simulink model "furuta_block_model_pi"  (R2026b)
settings: Solver=ode14x  StopTime=5  FixedStep=driveElectrical.sampleTime
model workspace (MAT data in the model file):
  controlPeriod = 0.01
  driveElectrical.R = 0.41
  driveElectrical.L = 0.00051
  driveElectrical.Ke = 1.73002596752
  driveElectrical.sampleTime = 0.0001
  driveElectrical.Kp = 0.480663675999
  driveElectrical.Ki = 386.415896392
  furutaPPOAgent : rl.agent.rlPPOAgent (value not decoded)
  furutaSACAgent : rl.agent.rlSACAgent (value not decoded)
  furutaToolboxMpc = mpc
  furutaToolboxMpc.Ts = 0.01
  furutaToolboxMpc.PredictionHorizon = 20
  furutaToolboxMpc.ControlHorizon = 20
  furutaToolboxMpc.Model.Plant = ss
  furutaToolboxMpc.Model.Plant.InputName_ = "MV1"
  furutaToolboxMpc.Model.Plant.InputGroup_.Manipulated = 1
  furutaToolboxMpc.Model.Plant.OutputName_ = ["MO1"; "MO2"; "MO3"; "MO4"; "MO5"; "MO6"; "MO7"; "MO8"]
  furutaToolboxMpc.Model.Plant.OutputGroup_.Measured = [1 2 3 4 5 6 7 8]
  furutaToolboxMpc.Model.Plant.IOSize_ = [8 1]
  furutaToolboxMpc.Model.Plant.Data_ = ltipack.ssdata
  furutaToolboxMpc.Model.Plant.Data_.a = [1  -0.00902674267589  0.00993774320897  -2.4767657698e-05; 0  1.0129802947  5.33054368483e-05  0.0100355972733; 0  -1.80504476453  0.987560350231  -0.00796081332398; 0  2.59780112786  0.0106592935191  1.01144622057]
  furutaToolboxMpc.Model.Plant.Data_.c = [1  0  0  0; 0  1  0  0; 0  0  1  0; 0  0  0  1; 23.187012799  50.483540443  3.96076595787  4.74600329341; 0  69.1342012244  4.52520194197  5.64653884547; 0  0  1.92549619263  1.610475723; 0  0  0  1.43133536407]
  furutaToolboxMpc.Model.Plant.Data_.dx0 = [0; 0; 0; 0]
  furutaToolboxMpc.Model.Plant.Data_.x0 = [0; 0; 0; 0]
  furutaToolboxMpc.Model.Plant.Data_.b = [0.0186770373086; -0.0159916310545; 3.73189493068; -3.19778805573]
  furutaToolboxMpc.Model.Plant.Data_.d = [0; 0; 0; 0; 0; 0; 0; 0]
  furutaToolboxMpc.Model.Plant.Data_.u0 = 0
  furutaToolboxMpc.Model.Plant.Data_.y0 = [0; 0; 0; 0; 0; 0; 0; 0]
  furutaToolboxMpc.Model.Plant.Data_.Delay.Input = 0
  furutaToolboxMpc.Model.Plant.Data_.Delay.Output = [0; 0; 0; 0; 0; 0; 0; 0]
  furutaToolboxMpc.Model.Plant.Data_.Delay.Internal = []
  furutaToolboxMpc.Model.Plant.Data_.Ts = 0.01
  furutaToolboxMpc.Model.Disturbance = []
  furutaToolboxMpc.Model.Noise = []
  furutaToolboxMpc.Model.Nominal.X = [0; 0; 0; 0]
  furutaToolboxMpc.Model.Nominal.DX = [0; 0; 0; 0]
  furutaToolboxMpc.Model.Nominal.U = 0
  furutaToolboxMpc.Model.Nominal.Y = [0; 0; 0; 0; 0; 0; 0; 0]
  furutaToolboxMpc.ManipulatedVariables.Min = [-1; -1; -1; -1; -1; -1; -1; -1; -1; -1; -1; -1; -1; -1; -1; -1; -1; -1; -1; -1]
  furutaToolboxMpc.ManipulatedVariables.Max = [1; 1; 1; 1; 1; 1; 1; 1; 1; 1; 1; 1; 1; 1; 1; 1; 1; 1; 1; 1]
  furutaToolboxMpc.ManipulatedVariables.MinECR = [0; 0; 0; 0; 0; 0; 0; 0; 0; 0; 0; 0; 0; 0; 0; 0; 0; 0; 0; 0]
  furutaToolboxMpc.ManipulatedVariables.MaxECR = [0; 0; 0; 0; 0; 0; 0; 0; 0; 0; 0; 0; 0; 0; 0; 0; 0; 0; 0; 0]
  furutaToolboxMpc.ManipulatedVariables.RateMin = -Inf
  furutaToolboxMpc.ManipulatedVariables.RateMax = Inf
  furutaToolboxMpc.ManipulatedVariables.RateMinECR = 0
  furutaToolboxMpc.ManipulatedVariables.RateMaxECR = 0
  furutaToolboxMpc.ManipulatedVariables.Target = 'nominal'
  furutaToolboxMpc.ManipulatedVariables.Name = 'MV1'
  furutaToolboxMpc.ManipulatedVariables.Units = ''
  furutaToolboxMpc.ManipulatedVariables.ScaleFactor = 1
  furutaToolboxMpc.ManipulatedVariables.Type = 'continuous'
  furutaToolboxMpc.OutputVariables(1).Min = [-Inf; -Inf; -Inf; -Inf; -Inf; -Inf; -Inf; -Inf; -Inf; -Inf; -Inf; -Inf; -Inf; -Inf; -Inf; -Inf; -Inf; -Inf; -Inf; -Inf]
  furutaToolboxMpc.OutputVariables(1).Max = [Inf; Inf; Inf; Inf; Inf; Inf; Inf; Inf; Inf; Inf; Inf; Inf; Inf; Inf; Inf; Inf; Inf; Inf; Inf; Inf]
  furutaToolboxMpc.OutputVariables(1).MinECR = [2; 2; 2; 2; 2; 2; 2; 2; 2; 2; 2; 2; 2; 2; 2; 2; 2; 2; 2; 2]
  furutaToolboxMpc.OutputVariables(1).MaxECR = [2; 2; 2; 2; 2; 2; 2; 2; 2; 2; 2; 2; 2; 2; 2; 2; 2; 2; 2; 2]
  furutaToolboxMpc.OutputVariables(1).Name = 'MO1'
  furutaToolboxMpc.OutputVariables(1).Units = ''
  furutaToolboxMpc.OutputVariables(1).ScaleFactor = 1
  furutaToolboxMpc.OutputVariables(2).Min = [-Inf; -Inf; -Inf; -Inf; -Inf; -Inf; -Inf; -Inf; -Inf; -Inf; -Inf; -Inf; -Inf; -Inf; -Inf; -Inf; -Inf; -Inf; -Inf; -Inf]
  furutaToolboxMpc.OutputVariables(2).Max = [Inf; Inf; Inf; Inf; Inf; Inf; Inf; Inf; Inf; Inf; Inf; Inf; Inf; Inf; Inf; Inf; Inf; Inf; Inf; Inf]
  furutaToolboxMpc.OutputVariables(2).MinECR = [2; 2; 2; 2; 2; 2; 2; 2; 2; 2; 2; 2; 2; 2; 2; 2; 2; 2; 2; 2]
  furutaToolboxMpc.OutputVariables(2).MaxECR = [2; 2; 2; 2; 2; 2; 2; 2; 2; 2; 2; 2; 2; 2; 2; 2; 2; 2; 2; 2]
  furutaToolboxMpc.OutputVariables(2).Name = 'MO2'
  furutaToolboxMpc.OutputVariables(2).Units = ''
  furutaToolboxMpc.OutputVariables(2).ScaleFactor = 1
  furutaToolboxMpc.OutputVariables(3).Min = [-Inf; -Inf; -Inf; -Inf; -Inf; -Inf; -Inf; -Inf; -Inf; -Inf; -Inf; -Inf; -Inf; -Inf; -Inf; -Inf; -Inf; -Inf; -Inf; -Inf]
  furutaToolboxMpc.OutputVariables(3).Max = [Inf; Inf; Inf; Inf; Inf; Inf; Inf; Inf; Inf; Inf; Inf; Inf; Inf; Inf; Inf; Inf; Inf; Inf; Inf; Inf]
  furutaToolboxMpc.OutputVariables(3).MinECR = [2; 2; 2; 2; 2; 2; 2; 2; 2; 2; 2; 2; 2; 2; 2; 2; 2; 2; 2; 2]
  furutaToolboxMpc.OutputVariables(3).MaxECR = [2; 2; 2; 2; 2; 2; 2; 2; 2; 2; 2; 2; 2; 2; 2; 2; 2; 2; 2; 2]
  furutaToolboxMpc.OutputVariables(3).Name = 'MO3'
  furutaToolboxMpc.OutputVariables(3).Units = ''
  furutaToolboxMpc.OutputVariables(3).ScaleFactor = 1
  furutaToolboxMpc.OutputVariables(4).Min = [-Inf; -Inf; -Inf; -Inf; -Inf; -Inf; -Inf; -Inf; -Inf; -Inf; -Inf; -Inf; -Inf; -Inf; -Inf; -Inf; -Inf; -Inf; -Inf; -Inf]
  furutaToolboxMpc.OutputVariables(4).Max = [Inf; Inf; Inf; Inf; Inf; Inf; Inf; Inf; Inf; Inf; Inf; Inf; Inf; Inf; Inf; Inf; Inf; Inf; Inf; Inf]
  furutaToolboxMpc.OutputVariables(4).MinECR = [2; 2; 2; 2; 2; 2; 2; 2; 2; 2; 2; 2; 2; 2; 2; 2; 2; 2; 2; 2]
  furutaToolboxMpc.OutputVariables(4).MaxECR = [2; 2; 2; 2; 2; 2; 2; 2; 2; 2; 2; 2; 2; 2; 2; 2; 2; 2; 2; 2]
  furutaToolboxMpc.OutputVariables(4).Name = 'MO4'
  furutaToolboxMpc.OutputVariables(4).Units = ''
  furutaToolboxMpc.OutputVariables(4).ScaleFactor = 1
  furutaToolboxMpc.OutputVariables(5).Min = [-Inf; -Inf; -Inf; -Inf; -Inf; -Inf; -Inf; -Inf; -Inf; -Inf; -Inf; -Inf; -Inf; -Inf; -Inf; -Inf; -Inf; -Inf; -Inf; -Inf]
  furutaToolboxMpc.OutputVariables(5).Max = [Inf; Inf; Inf; Inf; Inf; Inf; Inf; Inf; Inf; Inf; Inf; Inf; Inf; Inf; Inf; Inf; Inf; Inf; Inf; Inf]
  furutaToolboxMpc.OutputVariables(5).MinECR = [2; 2; 2; 2; 2; 2; 2; 2; 2; 2; 2; 2; 2; 2; 2; 2; 2; 2; 2; 2]
  furutaToolboxMpc.OutputVariables(5).MaxECR = [2; 2; 2; 2; 2; 2; 2; 2; 2; 2; 2; 2; 2; 2; 2; 2; 2; 2; 2; 2]
  furutaToolboxMpc.OutputVariables(5).Name = 'MO5'
  furutaToolboxMpc.OutputVariables(5).Units = ''
  furutaToolboxMpc.OutputVariables(5).ScaleFactor = 1
  furutaToolboxMpc.OutputVariables(6).Min = [-Inf; -Inf; -Inf; -Inf; -Inf; -Inf; -Inf; -Inf; -Inf; -Inf; -Inf; -Inf; -Inf; -Inf; -Inf; -Inf; -Inf; -Inf; -Inf; -Inf]
  furutaToolboxMpc.OutputVariables(6).Max = [Inf; Inf; Inf; Inf; Inf; Inf; Inf; Inf; Inf; Inf; Inf; Inf; Inf; Inf; Inf; Inf; Inf; Inf; Inf; Inf]
  furutaToolboxMpc.OutputVariables(6).MinECR = [2; 2; 2; 2; 2; 2; 2; 2; 2; 2; 2; 2; 2; 2; 2; 2; 2; 2; 2; 2]
  furutaToolboxMpc.OutputVariables(6).MaxECR = [2; 2; 2; 2; 2; 2; 2; 2; 2; 2; 2; 2; 2; 2; 2; 2; 2; 2; 2; 2]
  furutaToolboxMpc.OutputVariables(6).Name = 'MO6'
  furutaToolboxMpc.OutputVariables(6).Units = ''
  furutaToolboxMpc.OutputVariables(6).ScaleFactor = 1
  furutaToolboxMpc.OutputVariables(7).Min = [-Inf; -Inf; -Inf; -Inf; -Inf; -Inf; -Inf; -Inf; -Inf; -Inf; -Inf; -Inf; -Inf; -Inf; -Inf; -Inf; -Inf; -Inf; -Inf; -Inf]
  furutaToolboxMpc.OutputVariables(7).Max = [Inf; Inf; Inf; Inf; Inf; Inf; Inf; Inf; Inf; Inf; Inf; Inf; Inf; Inf; Inf; Inf; Inf; Inf; Inf; Inf]
  furutaToolboxMpc.OutputVariables(7).MinECR = [2; 2; 2; 2; 2; 2; 2; 2; 2; 2; 2; 2; 2; 2; 2; 2; 2; 2; 2; 2]
  furutaToolboxMpc.OutputVariables(7).MaxECR = [2; 2; 2; 2; 2; 2; 2; 2; 2; 2; 2; 2; 2; 2; 2; 2; 2; 2; 2; 2]
  furutaToolboxMpc.OutputVariables(7).Name = 'MO7'
  furutaToolboxMpc.OutputVariables(7).Units = ''
  furutaToolboxMpc.OutputVariables(7).ScaleFactor = 1
  furutaToolboxMpc.OutputVariables(8).Min = [-Inf; -Inf; -Inf; -Inf; -Inf; -Inf; -Inf; -Inf; -Inf; -Inf; -Inf; -Inf; -Inf; -Inf; -Inf; -Inf; -Inf; -Inf; -Inf; -Inf]
  furutaToolboxMpc.OutputVariables(8).Max = [Inf; Inf; Inf; Inf; Inf; Inf; Inf; Inf; Inf; Inf; Inf; Inf; Inf; Inf; Inf; Inf; Inf; Inf; Inf; Inf]
  furutaToolboxMpc.OutputVariables(8).MinECR = [2; 2; 2; 2; 2; 2; 2; 2; 2; 2; 2; 2; 2; 2; 2; 2; 2; 2; 2; 2]
  furutaToolboxMpc.OutputVariables(8).MaxECR = [2; 2; 2; 2; 2; 2; 2; 2; 2; 2; 2; 2; 2; 2; 2; 2; 2; 2; 2; 2]
  furutaToolboxMpc.OutputVariables(8).Name = 'MO8'
  furutaToolboxMpc.OutputVariables(8).Units = ''
  furutaToolboxMpc.OutputVariables(8).ScaleFactor = 1
  furutaToolboxMpc.Weights.ManipulatedVariables = [1; 1; 1; 1; 1; 1; 1; 1; 1; 1; 1; 1; 1; 1; 1; 1; 1; 1; 1; 1]
  furutaToolboxMpc.Weights.ManipulatedVariablesRate = 1e-05
  furutaToolboxMpc.Weights.OutputVariables = [3.16227766017  3.16227766017  1  1  0  0  0  0; 3.16227766017  3.16227766017  1  1  0  0  0  0; 3.16227766017  3.16227766017  1  1  0  0  0  0; 3.16227766017  3.16227766017  1  1  0  0  0  0; 3.16227766017  3.16227766017  1  1  0  0  0  0; 3.16227766017  3.16227766017  1  1  0  0  0  0; 3.16227766017  3.16227766017  1  1  0  0  0  0; 3.16227766017  3.16227766017  1  1  0  0  0  0; 3.16227766017  3.16227766017  1  1  0  0  0  0; 3.16227766017  3.16227766017  1  1  0  0  0  0; 3.16227766017  3.16227766017  1  1  0  0  0  0; 3.16227766017  3.16227766017  1  1  0  0  0  0; 3.16227766017  3.16227766017  1  1  0  0  0  0; 3.16227766017  3.16227766017  1  1  0  0  0  0; 3.16227766017  3.16227766017  1  1  0  0  0  0; 3.16227766017  3.16227766017  1  1  0  0  0  0; 3.16227766017  3.16227766017  1  1  0  0  0  0; 3.16227766017  3.16227766017  1  1  0  0  0  0; 3.16227766017  3.16227766017  1  1  0  0  0  0; 0  0  0  0  1  1  1  1]
  furutaToolboxMpc.Weights.ECR = 100000
  furutaToolboxMpc.Optimizer.OptimizationType = 'QP'
  furutaToolboxMpc.Optimizer.Solver = 'active-set'
  furutaToolboxMpc.Optimizer.SolverOptions = mpc.solver.options.qp.ActiveSet
  furutaToolboxMpc.Optimizer.SolverOptions.SolverName = 'ActiveSet'
  furutaToolboxMpc.Optimizer.MinOutputECR = 0
  furutaToolboxMpc.Optimizer.UseSuboptimalSolution = 0
  furutaToolboxMpc.Optimizer.CustomSolver = 0
  furutaToolboxMpc.Optimizer.CustomSolverCodeGen = 0
  furutaToolboxMpc.History = [2026 11 18 15 19 42.726]
  furutaToolboxMpc.MPCData = mpcdata
  furutaToolboxMpc.MPCData.IsDirty = 1
  furutaToolboxMpc.MPCData.Ts = 0.01
  furutaToolboxMpc.MPCData.p = 20
  furutaToolboxMpc.MPCData.m = 20
  furutaToolboxMpc.MPCData.UseActiveSetSolver = 1
  furutaToolboxMpc.MPCData.UseSuboptimalSolution = 0
  furutaToolboxMpc.MPCData.CustomSolver = 0
  furutaToolboxMpc.MPCData.CustomSolverCodeGen = 0
  furutaToolboxMpc.MPCData.IsCustomEstimation = 1
  furutaToolboxMpc.MPCData.Uscale = 1
  furutaToolboxMpc.MPCData.Yscale = [1; 1; 1; 1; 1; 1; 1; 1]
  furutaToolboxMpc.MPCData.mvindex = 1
  furutaToolboxMpc.MPCData.myindex = [1; 2; 3; 4; 5; 6; 7; 8]
  furutaToolboxMpc.MPCData.ASOptions.MaxIterations = 120
  furutaToolboxMpc.MPCData.ASOptions.MaxTime = Inf
  furutaToolboxMpc.MPCData.ASOptions.ConstraintTolerance = 1e-06
  furutaToolboxMpc.MPCData.ASOptions.UseWarmStart = 1
  furutaToolboxMpc.MPCData.IPOptions.MaxIterations = 50
  furutaToolboxMpc.MPCData.IPOptions.MaxTime = Inf
  furutaToolboxMpc.MPCData.IPOptions.ConstraintTolerance = 1e-06
  furutaToolboxMpc.MPCData.IPOptions.OptimalityTolerance = 1e-06
  furutaToolboxMpc.MPCData.IPOptions.ComplementarityTolerance = 1e-08
  furutaToolboxMpc.MPCData.IPOptions.StepTolerance = 1e-08
  furutaToolboxMpc.MPCData.ADOptions.AbsoluteTolerance = 0.001
  furutaToolboxMpc.MPCData.ADOptions.RelativeTolerance = 0.001
  furutaToolboxMpc.MPCData.ADOptions.MaxIterations = 1000
  furutaToolboxMpc.MPCData.ADOptions.MaxTime = Inf
  furutaToolboxMpc.MPCData.ADOptions.RelaxationParameter = 1.6
  furutaToolboxMpc.MPCData.ADOptions.PenaltyParameter = 0.1
  furutaToolboxMpc.MPCData.ADOptions.StepSize = 1e-06
  furutaToolboxMpc.MPCData.ADOptions.PrimalInfeasibilityTolerance = 0.0001
  furutaToolboxMpc.MPCData.ADOptions.DualInfeasibilityTolerance = 0.0001
  furutaToolboxMpc.MPCData.ADOptions.EnablePolish = 0
  furutaToolboxMpc.MPCData.ADOptions.PolishRegularization = 1e-06
  furutaToolboxMpc.MPCData.ADOptions.PolishTolerance = 1e-08
  furutaToolboxMpc.MPCData.ADOptions.PolishMaxIterations = 3
  furutaToolboxMpc.MPCData.MIQPOptions.MaxIterations = 1000
  furutaToolboxMpc.MPCData.MIQPOptions.MaxTime = Inf
  furutaToolboxMpc.MPCData.MIQPOptions.ConstraintTolerance = 1e-06
  furutaToolboxMpc.MPCData.MIQPOptions.UseWarmStart = 0
  furutaToolboxMpc.MPCData.MIQPOptions.DiscreteConstraintTolerance = 1e-06
  furutaToolboxMpc.MPCData.MIQPOptions.RoundingAtRootNode = 1
  furutaToolboxMpc.MPCData.MIQPOptions.MaxPendingNodes = 1000
  furutaToolboxMpc.IsEmpty = 0
  furutaToolboxMpc.OldOVIntegrator = {[]; []; []; []; []; []; []; []}
  furutaToolboxMpc.EstGain = 'custom'
  furutaToolboxMpc.OutDistModel = ss
  furutaToolboxMpc.OutDistModel.IOSize_ = [8 1]
  furutaToolboxMpc.OutDistModel.Data_ = ltipack.ssdata
  furutaToolboxMpc.OutDistModel.Data_.d = [0; 0; 0; 0; 0; 0; 0; 0]
  furutaToolboxMpc.OutDistModel.Data_.u0 = 0
  furutaToolboxMpc.OutDistModel.Data_.y0 = [0; 0; 0; 0; 0; 0; 0; 0]
  furutaToolboxMpc.OutDistModel.Data_.Delay.Input = 0
  furutaToolboxMpc.OutDistModel.Data_.Delay.Output = [0; 0; 0; 0; 0; 0; 0; 0]
  furutaToolboxMpc.OutDistModel.Data_.Delay.Internal = []
  furutaToolboxMpc.OutDistModel.Data_.Ts = 0
  furutaToolboxMpc.Version = '26.2'
  initialState = [0; 0.174532925199; 0; 0]
  integrationStep = 0.002
  lqrGain = [-0.560244322113 -7.30813603654 -0.304541725168 -0.68699829167]
  maxTorque = 0.03
  piReplayEnabled = 0
  piReplayState = [0  0  0  0  0; 5  0  0  0  0]
  pidGains = [7.30813603654 0.68699829167 0.560244322113 0.304541725168 0.01]
  plantCoefficients = [0.00019818 0.00016078 0.00016134 0.00013805 0.016934 0.0001 1e-05 0]
  rlRewardLevel = 2
  rmd.model = 'RMD-X6-P20-60-E'
  rmd.voltage = 48
  rmd.gearRatio = 19.612
  rmd.ratedTorque = 20
  rmd.ratedCurrent = 9.5
  rmd.ratedSpeedRPM = 153
  rmd.noLoadSpeedRPM = 176
  rmd.Kt = 2.1
  rmd.currentLSB = 0.01
  rmdCommandDelaySamples = 0
  scenarioStimulus = [0 0.0075 0.0175 0.0275 0.0375 0.0475 0.0575 0.0675 0.0775 0.0875 0.0975 0.1075 ... (2004 elements, 501x4)]
  usePolicyCallback = 0
  useRmd = 1
values from neighbouring files (symbols this model uses):
  C = [B A*B A^2*B A^3*B]    [build_furuta_rmd.m]
  N = 20    [build_furuta_rl.m]    (also in design_classical.m)
  s = load(matFile,'ds')    [analyze_pi_current_run.m]    (also in analyze_pi_speed_run.m; build_furuta_rl.m = sin(x(2));"; build_furuta_simulink.m = s(1); design_classical.m = furuta_scenarios)
  source = [step '/1']    [add_furuta_plant_blocks.m]    (also in build_furuta_pi.m = get_param(line,'SrcPortHandle'); build_furuta_pi_hardware.m = 'Drive interlocks/3'; compare_furuta_actuators.m = get_param([harness '/Requested torque'],'PortHandles'))
  Z = expm([A B; zeros(1,5)]*p.Ts)    [furuta_linearize.m]
undefined symbols (not defined in the file or in its folder): lmpcF, lmpcH, poleGain, sgn, X, Y
libraries: sm_lib x36, nesl_utility x8, fl_lib x7, rllib x2, mpclib x1, slpidlib x1, ee_lib x1
(part 1 of 4)
settings Model: Creator=Lsh  LastModifiedBy=Lsh
settings SimscapeCC: SimscapeLogType=all  SimscapeNominalValues="[{\"value\":\"1\",\"unit\":\"A\"},{\"value\":\"1\",\"unit\":\"bar\"},{\"value\":\"1\",\"unit\":\"cm^2\"},{\"value\":\"1\",\"unit\":\"cm^3/s\"},{\"value\":\"1\",\"unit\":\"kJ/kg\"},{\"value\":\"1\",\"unit\":\"kW\"},{\"value\":\"1\",\"unit\":\"l\"},{\"value\":\"1\",\"unit\":\"N\"},{\"value\":\"1\",\"unit\":\"N*m\"},{\"value\":\"1\",\"unit\":\"V\"},{\"value\":\"0.001\",\"unit\":\"Wb\"}]"  SimscapeUseEnergyAccounting=off

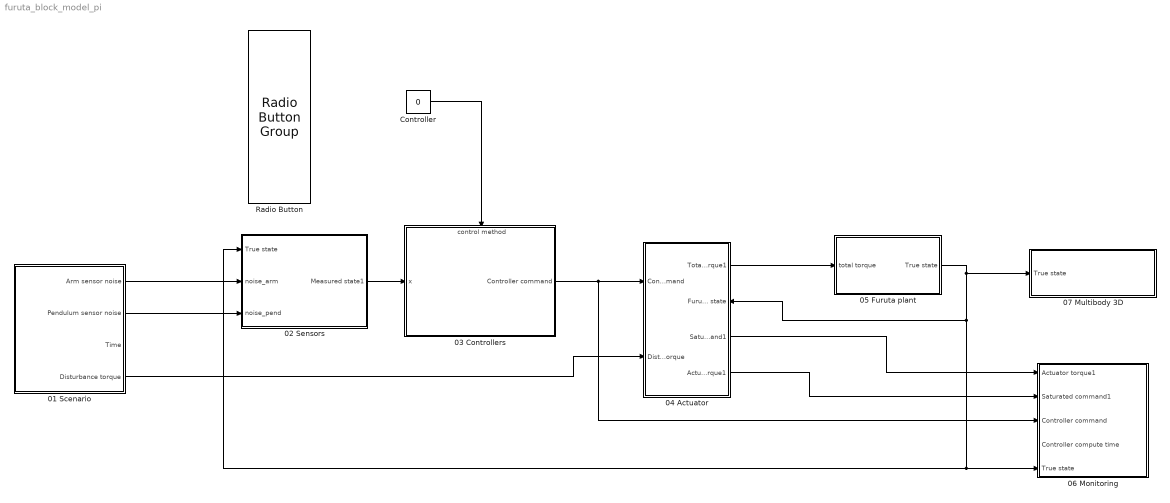
== system furuta_block_model_pi ==
  01 Scenario : Subsystem
  02 Sensors : Subsystem
  03 Controllers : Subsystem
      settings: PortSchema="{\"entries\":[{\"content\":{\"sides\":[{\"content\":{\"connectorIds\":[\"In1\"]},\"type\":\"ConnectorPlacement.EquallySpacedRectSide\",\"uuid\":\"e4b36115-6a1d-4962-9ef8-ed5f31cfcc6a\"},{\"content\":{\"connectorIds\":[\"Out1\"],\"side\":\"RIGHT\"},\"type\":\"ConnectorPlacement.EquallySpacedRectSide\",\"uuid\":\"30852384-c2a0-433b-a443-149c1bfb4c73\"},{\"content\":{\"connectorIds\":[\"In2\"],\"side\":\"TOP\"},\"type\":\"ConnectorPlacement.EquallySpacedRectSide\",\"uuid\":\"d3eba7d3-47d6-4151-b089-0f7eaff5c42c\"},{\"content\":{\"side\":\"BOTTOM\"},\"type\":\"ConnectorPlacement.EquallySpacedRectSide\",\"uuid\":\"8130c781-304c-497e-8c63-b3eca62ccf99\"}]},\"type\":\"ConnectorPlacement.EquallySpacedConnector\",\"uuid\":\"c7c0857b-c1c9-4543-82a8-21998e0f16d7\"}],\"packageUris\":[\"http://schema.mathworks.com/mf0/Connector/R2020b\"],\"version\":\"1.0\"}"
  04 Actuator : Subsystem
      settings: PortSchema="{\"entries\":[{\"content\":{\"sides\":[{\"content\":{\"connectorIds\":[\"In1\",\"In2\"]},\"type\":\"ConnectorPlacement.EquallySpacedRectSide\",\"uuid\":\"dd482a63-174b-40e1-9b64-24dbfdc3f8fa\"},{\"content\":{\"connectorIds\":[\"Out1\",\"In3\",\"Out2\",\"Out3\"],\"side\":\"RIGHT\"},\"type\":\"ConnectorPlacement.EquallySpacedRectSide\",\"uuid\":\"33c1ee09-a2ec-4fc3-8e05-903f6e1c4f35\"},{\"content\":{\"side\":\"TOP\"},\"type\":\"ConnectorPlacement.EquallySpacedRectSide\",\"uuid\":\"197082e8-1213-404b-be05-6b5ef49382e8\"}]},\"type\":\"ConnectorPlacement.EquallySpacedConnector\",\"uuid\":\"93af0a87-d82b-49a5-b998-c75b367beb5b\"}],\"packageUris\":[\"http://schema.mathworks.com/mf0/Connector/R2020b\"],\"version\":\"1.0\"}"
  05 Furuta plant : Subsystem
  06 Monitoring : Subsystem
  07 Multibody 3D : Subsystem
  Controller : Constant  Value=0
  Radio Button : RadioButtonGroup  SelectedLabel=PID  ButtonGroupName=Group
  wires:
  01 Scenario/1(Arm sensor noise) -> 02 Sensors/2(noise_arm)
  01 Scenario/2(Pendulum sensor noise) -> 02 Sensors/3(noise_pend)
  03 Controllers/1(Controller command) -> 06 Monitoring/3(Controller command), 04 Actuator/1(Controller command)
  02 Sensors/1(Measured state1) -> 03 Controllers/1(x)
  01 Scenario/4(Disturbance torque) -> 04 Actuator/2(Disturbance torque)
  05 Furuta plant/1(True state) -> 02 Sensors/1(True state), 06 Monitoring/5(True state), 04 Actuator/3(Furuta state), 07 Multibody 3D/1(True state)
  04 Actuator/1(Total torque1) -> 05 Furuta plant/1(total torque)
  04 Actuator/2(Saturated command1) -> 06 Monitoring/1(Actuator torque1)
  04 Actuator/3(Actuator torque1) -> 06 Monitoring/2(Saturated command1)
  Controller/1 -> 03 Controllers/2(control method)

== system furuta_block_model_pi/01 Scenario ==
  Clock : DigitalClock  SampleTime=controlPeriod
  Scenario : FromWorkspace  VariableName=scenarioStimulus  SampleTime=controlPeriod  Interpolate=off  OutputAfterFinalValue=Holding final value
  Scenario channels : Demux  Outputs=3
  Arm sensor noise : Outport
  Pendulum sensor noise : Outport  Port=2
  Time : Outport  Port=3
  Disturbance torque : Outport  Port=4
  wires:
  Scenario channels/1 -> Arm sensor noise/1  "Arm sensor noise"
  Clock/1 -> Time/1  "Time"
  Scenario/1 -> Scenario channels/1
  Scenario channels/3 -> Disturbance torque/1  "Disturbance torque"
  Scenario channels/2 -> Pendulum sensor noise/1  "Pendulum sensor noise"

== system furuta_block_model_pi/02 Sensors ==
  True state : Inport
  noise_arm : Inport  Port=2
  noise_pend : Inport  Port=3
  Measured arm : Sum
  Measured pendulum : Sum
  Measured state : Mux
  State channels : Demux
  Measured state1 : Outport
  wires:
  True state/1 -> State channels/1
  State channels/1 -> Measured arm/1  "Arm angle"
  Measured state/1 -> Measured state1/1  "Measured state"
  State channels/2 -> Measured pendulum/1  "Pendulum angle"
  Measured arm/1 -> Measured state/1
  Measured pendulum/1 -> Measured state/2
  State channels/4 -> Measured state/4
  State channels/3 -> Measured state/3
  noise_arm/1 -> Measured arm/2
  noise_pend/1 -> Measured pendulum/2

== system furuta_block_model_pi/03 Controllers ==
  x : Inport
  control method : Inport  Port=2
  Controller bank : MultiPortSwitch  DataPortOrder=Zero-based contiguous  Inputs=5  zeroidx=on  SaturateOnIntegerOverflow=off  InputSameDT=off
  LMPC (sim) : Subsystem  Commented=on
  LQR : Subsystem
  MPC Controller : Subsystem
  PID : Subsystem
  PPO : Subsystem
  Pendulum and arm PD : Subsystem  Commented=on
  Pole placement : Subsystem  Commented=on
  SAC : Subsystem
  Controller command : Outport
  wires:
  PPO/1(Out1) -> Controller bank/5
  control method/1 -> PID/1(mode), SAC/2(mode), PPO/1(Controller mode), LQR/1(mode), Controller bank/1
  LQR/1(u) -> Controller bank/3
  Controller bank/1 -> Controller command/1
  PID/1(u) -> Controller bank/2
  MPC Controller/1(mv) -> Controller bank/4
  x/1 -> SAC/1(x), PPO/2(Measured state), PID/2(x), LQR/2(x), MPC Controller/1(mo or x)
  SAC/1(Out1) -> Controller bank/6

== system furuta_block_model_pi/04 Actuator ==
  note: Parameters
      | RMD-X6-P20-60-E
      |
      | Gear Ratio
      | 19.612
      |
      | Input Voltage (V)
      | 48
      |
      | No Load Speed (RPM)
      | 176
      |
      | No Load Input Current (A)
      | 0.9
      |
      | Rated Speed (RPM)
      | 153
      |
      | Rated Torque (N·m)
      | 20
      |
      | Rated Output Power (W)
      | 320
      |
      | Rated Phase Current
      | 9.5
      |
      | (A rms)
      |
      | Peak Torque (N·m)
      | 60
      |
      | Peak Phase Current
      | 29.1
      |
      | (A rms)
      |
      | Efficiency (%)
      | 72.7
      |
      | Motor Back-EMF Constant (Vdc/Krpm)
      | 16
      |
      | Module Torque Constant (N·m/A)
      | 2.1
      |
      | Motor Phase Resistance (Ω)
      | 0.41
      |
      | Motor Phase Inductance (mH)
      | 0.51
      |
      | Pole Pair
      | 10
      |
      | 3 Phase Connection
      | Y
      |
      | Back Drive Torque (N·m)
      | 1.6
      |
      | Backlash (Arcmin)
      | 10
      |
      | Output Bearing Type
      | Crossed Roller Bearings
      |
      | Axial Load - Tension (kN)
      | 1.8
      |
      | Axial Load - Compression (kN)
      | 0.8
      |
      | Radial Load (kN)
      | 2
      |
      | Inertia (Kg·cm²)
      | 0.66
      |
      | Dual Encoder Type & Interface
      | ABS-17BIT (Input) / 17BIT (Output)
      |
      | Repeat Position Accuracy (°)
      | < 0.01
      |
      | Communication
      | EtherCAT
      |
      | Weight (kg)
      | 0.82
      |
      | Insulation Grade
      | F
  Controller command : Inport
  Disturbance torque : Inport  Port=2
  Furuta state : Inport  Port=3
  Actuator limits1 : Saturate  UpperLimit=1  LowerLimit=-1
  Add disturbance1 : Sum
  Applied torque log : ToWorkspace  VariableName=appliedTorqueTrace  SampleTime=-1
  Extract arm speed : Fcn  Expr=u(3)
  RMD X6 P20 60 E : Subsystem
  Select actuator : Switch  Threshold=0.5  SaturateOnIntegerOverflow=off  InputSameDT=off
  Torque Nm1 : Gain  Gain=maxTorque
  Use RMD : Constant  Value=useRmd
  Total torque1 : Outport
  Saturated command1 : Outport  Port=2
  Actuator torque1 : Outport  Port=3
  wires:
  Disturbance torque/1 -> Add disturbance1/2
  Torque Nm1/1 -> Select actuator/3, RMD X6 P20 60 E/2(Requested torque)  "Actuator torque"
  Furuta state/1 -> Extract arm speed/1
  Use RMD/1 -> Select actuator/2
  Controller command/1 -> Actuator limits1/1
  Extract arm speed/1 -> RMD X6 P20 60 E/1(Output shaft speed)
  Actuator limits1/1 -> Torque Nm1/1, Saturated command1/1  "Saturated command"
  RMD X6 P20 60 E/1(Output torque) -> Select actuator/1
  Select actuator/1 -> Actuator torque1/1, Add disturbance1/1, Applied torque log/1
  Add disturbance1/1 -> Total torque1/1  "Total torque"

== system furuta_block_model_pi/05 Furuta plant ==
  total torque : Inport
  Plant state : UnitDelay  InitialCondition=initialState  SampleTime=controlPeriod
  RK4 Furuta plant : Subsystem
  True state : Outport
  wires:
  RK4 Furuta plant/1(next state) -> Plant state/1
  Plant state/1 -> True state/1, RK4 Furuta plant/1(state)  "True state"
  total torque/1 -> RK4 Furuta plant/2(total torque)

== system furuta_block_model_pi/06 Monitoring ==
  Actuator torque1 : Inport
  Saturated command1 : Inport  Port=2
  Controller command : Inport  Port=3
  Controller compute time : Inport  Port=4
  True state : Inport  Port=5
  Action log : ToWorkspace  VariableName=actionTrace  SampleTime=-1
  Angle signals : Mux  Inputs=2
  Arm and pendulum : Scope
  Arm deg : Gain  Gain=180/pi
  Command log : ToWorkspace  VariableName=commandTrace  SampleTime=-1
  Compute log : ToWorkspace  VariableName=computeTrace  SampleTime=-1
  Control torque : Scope
  Pendulum deg : Fcn  Expr=atan2(sin(u),cos(u))*180/pi
  State channels : Demux
  State log : ToWorkspace  VariableName=stateTrace  SampleTime=-1
  wires:
  Controller command/1 -> Command log/1
  True state/1 -> State log/1, State channels/1
  Controller compute time/1 -> Compute log/1
  Saturated command1/1 -> Control torque/1
  Actuator torque1/1 -> Action log/1
  Angle signals/1 -> Arm and pendulum/1
  Pendulum deg/1 -> Angle signals/2
  Arm deg/1 -> Angle signals/1
  State channels/1 -> Arm deg/1  "Arm angle"
  State channels/2 -> Pendulum deg/1  "Pendulum angle"
